simulink model "MD_sfunc_test_3dof_opfFrc_2024a"  (R2024a)
settings: Solver=FixedStepDiscrete  StartTime=0.0  StopTime=TMax  FixedStep=dt  RelTol=1e-3
settings Model: Creator=Andreas  LastModifiedBy=Andreas
settings ConfigComp: CovBoundaryAbsTol=1.0e-5

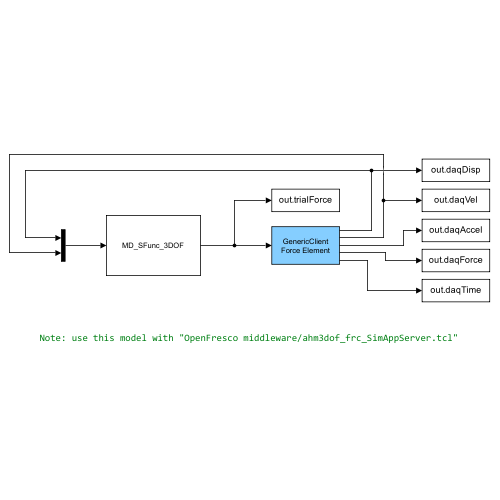
[thumbnail: Simulink's stored preview of the top-level diagram]
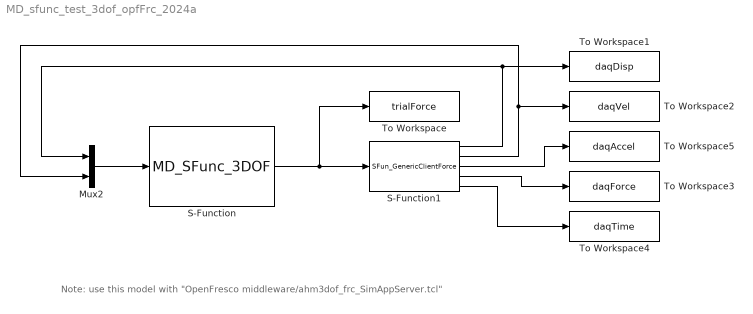
== system MD_sfunc_test_3dof_opfFrc_2024a ==
  note: Note: use this model with "OpenFresco middleware/ahm3dof_frc_SimAppServer.tcl"
  Mux2 : Mux  Inputs=2
  S-Function : S-Function  FunctionName=MD_SFunc_3DOF  Parameters=MD_InputFileName, dt, TMax  SFunctionDeploymentMode=off  EnableBusSupport=off
  S-Function1 : S-Function  FunctionName=SFun_GenericClientForce  Parameters=ipAddr,ipPort,dataSize  SFunctionDeploymentMode=off  EnableBusSupport=off  mask(GenericClient Element){ipAddr=127.0.0.1, ipPort=8090, dataSize=256}
      mask prompts: ipAddr "IP Address of Server"; ipPort "IP Port Number of Server"; dataSize "Size of Data Arrays"
      mask Display: disp('GenericClient\nForce Element');
  To Workspace : ToWorkspace  VariableName=trialForce  SaveFormat=Timeseries  SampleTime=-1
  To Workspace1 : ToWorkspace  VariableName=daqDisp  SaveFormat=Timeseries  SampleTime=-1
  To Workspace2 : ToWorkspace  VariableName=daqVel  SaveFormat=Timeseries  SampleTime=-1
  To Workspace3 : ToWorkspace  VariableName=daqForce  SaveFormat=Timeseries  SampleTime=-1
  To Workspace4 : ToWorkspace  VariableName=daqTime  SaveFormat=Timeseries  SampleTime=-1
  To Workspace5 : ToWorkspace  VariableName=daqAccel  SaveFormat=Timeseries  SampleTime=-1
  wires:
  S-Function/1 -> To Workspace/1, S-Function1/1
  S-Function1/1 -> Mux2/1, To Workspace1/1
  S-Function1/2 -> Mux2/2, To Workspace2/1
  S-Function1/4 -> To Workspace3/1
  S-Function1/5 -> To Workspace4/1
  S-Function1/3 -> To Workspace5/1
  Mux2/1 -> S-Function/1
